simulink model "YMBOX_Control_Core"  (R2024b)
settings: Solver=FixedStepDiscrete  StartTime=0.0  StopTime=3  RelTol=1e-3
PreLoadFcn:
  | run(fullfile(fileparts(get_param(bdroot,'FileName')), 'YMBOX_Deluxe_init.m'));
InitFcn:
  | YMBOX_InitializeModel('core',bdroot);
model workspace (MAT data in the model file):
  KuMDAS_ObserverBuildVariant : Simulink.Parameter (value not decoded)
undefined symbols (not defined in the file or in its folder): CeMDSM_DrvModeIfStart_enum, CeMDSM_DrvModeSpdSens_enum, CeMDSM_DrvModeSpdSmo_enum, CeMDSM_DrvModeTrq_enum, Cf_CONTROL_TASK_TIME_S, KbMDAS_SmoDeadTimeCompEnable_flg, KbMDSA_ActiveInverterCompEnable_flg, KbMDSA_UnifiedVoltageLimitEnable_flg, KbMDSP_DCBusVoltReportFilterEnable_flg, KbMDTM_DAxisPriorityInFW_flg, KbMDTM_FieldWeakeningEnable_flg, KbMDTM_FinalIqAntiWindupEnable_flg, KbMDTM_SensorlessFieldWeakeningEnable_flg, KbMDTM_TorquePriorityBelowBase_flg, KbMDTM_UnifiedConstraintEnable_flg, KfMDAS_ControlCountToElecRad_NULL, KfMDAS_IfAccel_rpms, KfMDAS_IfAlignTime_s, KfMDAS_IfBlendTime_s, KfMDAS_IfSwitchSpd_rpm, KfMDAS_NativeCountToMechRad_NULL, KfMDAS_ObserverExitRatio_NULL, KfMDAS_SlsCtrlPeriod_s, KfMDAS_SlsEAngleInit_rad, KfMDAS_SlsElecSpdMax_rads, KfMDAS_SlsElecSpdMin_rads, KfMDAS_SlsTwoPi_rad, KfMDAS_SmoAngleOffset_rad, KfMDAS_SmoCurrentZohCoefA_NULL, KfMDAS_SmoCurrentZohCoefB_AperV, KfMDAS_SmoDeadTimeCurrentBoundary_A, KfMDAS_SmoDeadTimeDuty_NULL, KfMDAS_SmoDeadTimePolarity_NULL, KfMDAS_SmoDeviceDrop_V, KfMDAS_SmoEmfLpfCoefA_NULL, KfMDAS_SmoEmfLpfCoefB_NULL, KfMDAS_SmoEmfLpfInvPole_s, KfMDAS_SmoErrBoundaryMax_A, KfMDAS_SmoErrBoundarySpan_A, KfMDAS_SmoGainSchedAlpha_NULL, KfMDAS_SmoGainSchedAngleComp_rad, KfMDAS_SmoGainSchedEmfLow_V, KfMDAS_SmoGainSchedInvSpan_PerV, KfMDAS_SmoLdMinusLq_H, KfMDAS_SmoPllKiTs_NULL, KfMDAS_SmoPllKp_NULL, KfMDAS_SmoPllMinEmf_V, KfMDAS_SmoPllSpeedLpfAlpha_NULL, KfMDAS_SmoSlideGainMin_V, KfMDAS_SmoSlideGainSpan_V, KfMDAS_SmoSwitchSpd_rpm, KfMDAS_SmoTotalDelay_s, KfMDCC_DqSoftwareOverCurrentThreshold_A, KfMDCC_PiKcTsId_NULL, KfMDCC_PiKcTsIq_NULL, KfMDCC_PiKiTsId_NULL, KfMDCC_PiKiTsIq_NULL, KfMDCC_PiKpValueId_NULL, KfMDCC_PiKpValueIq_NULL, KfMDCC_PwmFreq_Hz ... (+84)
libraries: YMBOX_SharedMath_Lib x11, spsabctoAlphaBetaZeroLib x1
(part 5 of 8)

== system YMBOX_Control_Core/MDAS/Sensorless_FluxMRAS/Observer_Variant1_SMO/Voltage_AlphaBeta_Reconstruction ==
  VfMDAS_SlsPwmDutyPhaseU_NULL : Inport
  VfMDAS_SlsPwmDutyPhaseV_NULL : Inport  Port=2
  VfMDAS_SlsPwmDutyPhaseW_NULL : Inport  Port=3
  PhaseCurrentU_A : Inport  Port=4
  PhaseCurrentV_A : Inport  Port=5
  PhaseCurrentW_A : Inport  Port=6
  DcBusVoltage_V : Inport  Port=7
  CurrentSignSatU : Saturate  UpperLimit=1  LowerLimit=-1
  CurrentSignSatV : Saturate  UpperLimit=1  LowerLimit=-1
  CurrentSignSatW : Saturate  UpperLimit=1  LowerLimit=-1
  CurrentSignU : Gain  Gain=1/KfMDAS_SmoDeadTimeCurrentBoundary_A
  CurrentSignV : Gain  Gain=1/KfMDAS_SmoDeadTimeCurrentBoundary_A
  CurrentSignW : Gain  Gain=1/KfMDAS_SmoDeadTimeCurrentBoundary_A
  DeadTimeDuty : Gain  Gain=KfMDAS_SmoDeadTimeDuty_NULL
  DeadTimeEnablePolarity : Gain  Gain=KbMDAS_SmoDeadTimeCompEnable_flg*KfMDAS_SmoDeadTimePolarity_NULL
  DeadTimeErrorU : Product  Inputs=**  OutDataTypeStr=single  RndMeth=Nearest  SaturateOnIntegerOverflow=on
  DeadTimeErrorV : Product  Inputs=**  OutDataTypeStr=single  RndMeth=Nearest  SaturateOnIntegerOverflow=on
  DeadTimeErrorW : Product  Inputs=**  OutDataTypeStr=single  RndMeth=Nearest  SaturateOnIntegerOverflow=on
  DeadTimeVoltage : Sum  OutDataTypeStr=single  AccumDataTypeStr=single  RndMeth=Nearest  SaturateOnIntegerOverflow=on
  DeviceDrop : Constant  Value=KfMDAS_SmoDeviceDrop_V  OutDataTypeStr=single
  Duty_alpha_sum : Sum  Inputs=+--
  Duty_beta_sum : Sum  Inputs=+-
  ErrorAlpha : Gain  Gain=2/3
  ErrorAlphaRaw : Sum  Inputs=+--  OutDataTypeStr=single  AccumDataTypeStr=single  RndMeth=Nearest  SaturateOnIntegerOverflow=on
  ErrorBeta : Gain  Gain=sqrt(3)/3
  ErrorBetaRaw : Sum  Inputs=+-  OutDataTypeStr=single  AccumDataTypeStr=single  RndMeth=Nearest  SaturateOnIntegerOverflow=on
  HalfErrorV : Gain  Gain=0.5
  HalfErrorW : Gain  Gain=0.5
  Half_Duty_V : Gain  Gain=0.5
  Half_Duty_W : Gain  Gain=0.5
  Mux_Uab0 : Mux  Inputs=3
  UalphaCompensated : Sum  Inputs=+-  OutDataTypeStr=single  AccumDataTypeStr=single  RndMeth=Nearest  SaturateOnIntegerOverflow=on
  Ualpha_gain : Gain  Gain=2/3
  Ualpha_single : DataTypeConversion  OutDataTypeStr=single  SaturateOnIntegerOverflow=off  RndMeth=Floor
  UbetaCompensated : Sum  Inputs=-+  OutDataTypeStr=single  AccumDataTypeStr=single  RndMeth=Nearest  SaturateOnIntegerOverflow=on
  Ubeta_gain : Gain  Gain=sqrt(3)/3
  Ubeta_single : DataTypeConversion  OutDataTypeStr=single  SaturateOnIntegerOverflow=off  RndMeth=Floor
  VdcDutyAlpha : Product  Inputs=**  OutDataTypeStr=single  RndMeth=Nearest  SaturateOnIntegerOverflow=on
  VdcDutyBeta : Product  Inputs=**  OutDataTypeStr=single  RndMeth=Nearest  SaturateOnIntegerOverflow=on
  Zero_Sequence : Constant  Value=single(0)  OutDataTypeStr=single
  VfMDAS_SlsVoltAlphaBetaZero_V : Outport
  wires:
  Half_Duty_W/1 -> Duty_alpha_sum/3
  Duty_alpha_sum/1 -> VdcDutyAlpha/1
  ErrorAlpha/1 -> UalphaCompensated/2
  VfMDAS_SlsPwmDutyPhaseV_NULL/1 -> Half_Duty_V/1, Duty_beta_sum/1
  DeadTimeErrorV/1 -> HalfErrorV/1, ErrorBetaRaw/1
  DcBusVoltage_V/1 -> VdcDutyBeta/1, DeadTimeDuty/1, VdcDutyAlpha/2
  Mux_Uab0/1 -> VfMDAS_SlsVoltAlphaBetaZero_V/1
  VfMDAS_SlsPwmDutyPhaseU_NULL/1 -> Duty_alpha_sum/1
  DeadTimeEnablePolarity/1 -> DeadTimeErrorU/2, DeadTimeErrorW/1, DeadTimeErrorV/1
  VfMDAS_SlsPwmDutyPhaseW_NULL/1 -> Half_Duty_W/1, Duty_beta_sum/2
  Duty_beta_sum/1 -> VdcDutyBeta/2
  VdcDutyAlpha/1 -> Ualpha_gain/1
  Half_Duty_V/1 -> Duty_alpha_sum/2
  ErrorAlphaRaw/1 -> ErrorAlpha/1
  Ualpha_gain/1 -> UalphaCompensated/1
  PhaseCurrentU_A/1 -> CurrentSignU/1
  DeadTimeErrorU/1 -> ErrorAlphaRaw/1
  PhaseCurrentV_A/1 -> CurrentSignV/1
  DeadTimeDuty/1 -> DeadTimeVoltage/1
  DeviceDrop/1 -> DeadTimeVoltage/2
  VdcDutyBeta/1 -> Ubeta_gain/1
  ErrorBeta/1 -> UbetaCompensated/1
  PhaseCurrentW_A/1 -> CurrentSignW/1
  CurrentSignU/1 -> CurrentSignSatU/1
  CurrentSignV/1 -> CurrentSignSatV/1
  HalfErrorW/1 -> ErrorAlphaRaw/3
  DeadTimeVoltage/1 -> DeadTimeEnablePolarity/1
  CurrentSignW/1 -> CurrentSignSatW/1
  CurrentSignSatU/1 -> DeadTimeErrorU/1
  CurrentSignSatV/1 -> DeadTimeErrorV/2
  CurrentSignSatW/1 -> DeadTimeErrorW/2
  DeadTimeErrorW/1 -> HalfErrorW/1, ErrorBetaRaw/2
  Ubeta_gain/1 -> UbetaCompensated/2
  HalfErrorV/1 -> ErrorAlphaRaw/2
  ErrorBetaRaw/1 -> ErrorBeta/1
  UbetaCompensated/1 -> Ubeta_single/1
  UalphaCompensated/1 -> Ualpha_single/1
  Ubeta_single/1 -> Mux_Uab0/2
  Ualpha_single/1 -> Mux_Uab0/1
  Zero_Sequence/1 -> Mux_Uab0/3

== system YMBOX_Control_Core/MDCC/MDCC_Subsystem/DqSoftwareOverCurrent_Diagnostic/CountWhenDqCurrentExceeded ==
  VuMDCC_DqSoftwareOverCurrentCount_cnt : Inport  OutDataTypeStr=uint8
  Action Port : ActionPort  ActionPortLabel=if(u1 > u2 | u1 ~= u1)
  AssertDqSoftwareOverCurrent : Subsystem  TreatAsAtomicUnit=on
  DqSoftwareOverCurrentConfirmCount : Constant  Value=KuMDCC_DqSoftwareOverCurrentConfirm_cnt
  If : If  NumInputs=2  IfExpression=u1<u2
  IncrementDqSoftwareOverCurrentCount : Subsystem  TreatAsAtomicUnit=on
  VbMDCC_DqSoftwareOverCurrent_flg : Outport  OutputWhenDisabled=reset  InitialOutput=false
  VuMDCC_DqSoftwareOverCurrentCountNew_cnt : Outport  Port=2
  wires:
  DqSoftwareOverCurrentConfirmCount/1 -> If/2
  If/1 -> IncrementDqSoftwareOverCurrentCount/Action
  If/2 -> AssertDqSoftwareOverCurrent/Action
  IncrementDqSoftwareOverCurrentCount/1(VuMDCC_DqSoftwareOverCurrentCountNew_cnt) -> VuMDCC_DqSoftwareOverCurrentCountNew_cnt/1
  AssertDqSoftwareOverCurrent/1(VbMDCC_DqSoftwareOverCurrent_flg) -> VbMDCC_DqSoftwareOverCurrent_flg/1
  VuMDCC_DqSoftwareOverCurrentCount_cnt/1 -> IncrementDqSoftwareOverCurrentCount/1(VuMDCC_DqSoftwareOverCurrentCount_cnt), If/1

== system YMBOX_Control_Core/MDCC/MDCC_Subsystem/DqSoftwareOverCurrent_Diagnostic/CountWhenDqCurrentNormal ==
  VuMDCC_DqSoftwareOverCurrentCount_cnt : Inport
  Action Port : ActionPort  ActionPortLabel=else
  DecrementDqSoftwareOverCurrentCount : Subsystem  TreatAsAtomicUnit=on
  If : If  IfExpression=u1~=0  ShowElse=off
  VuMDCC_DqSoftwareOverCurrentCountNew_cnt : Outport
  wires:
  DecrementDqSoftwareOverCurrentCount/1(VuMDCC_DqSoftwareOverCurrentCountNew_cnt) -> VuMDCC_DqSoftwareOverCurrentCountNew_cnt/1
  If/1 -> DecrementDqSoftwareOverCurrentCount/Action
  VuMDCC_DqSoftwareOverCurrentCount_cnt/1 -> If/1, DecrementDqSoftwareOverCurrentCount/1(VuMDCC_DqSoftwareOverCurrentCount_cnt)

== system YMBOX_Control_Core/MDCC/MDCC_Subsystem/DqSoftwareOverCurrent_Diagnostic/Current_Magnitude_Squared ==
  VfMDCC_DCur_A : Inport
  VfMDCC_QCur_A : Inport  Port=2
  Product : Product
  Product1 : Product
  Sum : Sum
  VfMDCC_CurMagnitudeSq_A2 : Outport
  wires:
  VfMDCC_QCur_A/1 -> Product1/2, Product1/1
  VfMDCC_DCur_A/1 -> Product/1, Product/2
  Product1/1 -> Sum/2
  Product/1 -> Sum/1
  Sum/1 -> VfMDCC_CurMagnitudeSq_A2/1  "VfMDCC_CurMagnitudeSq_A2"

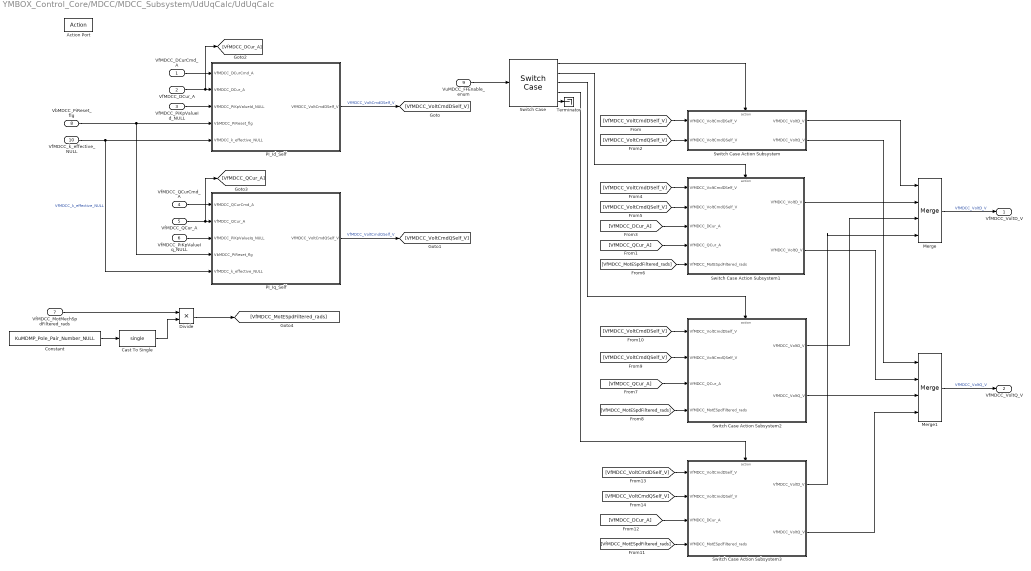
== system YMBOX_Control_Core/MDCC/MDCC_Subsystem/UdUqCalc/UdUqCalc ==
  VfMDCC_DCurCmd_A : Inport
  VfMDCC_DCur_A : Inport  Port=2
  VfMDCC_PiKpValueId_NULL : Inport  Port=3
  VfMDCC_QCurCmd_A : Inport  Port=4
  VfMDCC_QCur_A : Inport  Port=5
  VfMDCC_PiKpValueIq_NULL : Inport  Port=6
  VfMDCC_MotMechSpdFiltered_rads : Inport  Port=7
  VbMDCC_PiReset_flg : Inport  Port=8
  VuMDCC_FFEnable_enum : Inport  Port=9
  VfMDCC_k_effective_NULL : Inport  Port=10
  Action Port : ActionPort  ActionPortLabel=default:
  Cast To Single : DataTypeConversion  OutDataTypeStr=single  SaturateOnIntegerOverflow=off  RndMeth=Floor
  Constant : Constant  Value=KuMDMP_Pole_Pair_Number_NULL
  Divide : Product  Inputs=**
  Merge : Merge  Inputs=4
  Merge1 : Merge  Inputs=4
  PI_Id_Self : Subsystem
  PI_Iq_Self : Subsystem
  Switch Case : SwitchCase  CaseConditions={0,1,2,3}
  Switch Case Action Subsystem : Subsystem  TreatAsAtomicUnit=on
  Switch Case Action Subsystem1 : Subsystem  TreatAsAtomicUnit=on
  Switch Case Action Subsystem2 : Subsystem  TreatAsAtomicUnit=on
  Switch Case Action Subsystem3 : Subsystem  TreatAsAtomicUnit=on
  Terminator : Terminator
  VfMDCC_VoltD_V : Outport
  VfMDCC_VoltQ_V : Outport  Port=2
  wires:
  Cast To Single/1 -> Divide/2
  Constant/1 -> Cast To Single/1
  VfMDCC_MotMechSpdFiltered_rads/1 -> Divide/1
  Divide/1 -> [VfMDCC_MotESpdFiltered_rads]
  [VfMDCC_MotESpdFiltered_rads] -> Switch Case Action Subsystem2/4(VfMDCC_MotESpdFiltered_rads)
  [VfMDCC_MotESpdFiltered_rads] -> Switch Case Action Subsystem1/5(VfMDCC_MotESpdFiltered_rads)
  Switch Case/4 -> Switch Case Action Subsystem3/Action
  Switch Case/3 -> Switch Case Action Subsystem2/Action
  Switch Case/2 -> Switch Case Action Subsystem1/Action
  Switch Case/1 -> Switch Case Action Subsystem/Action
  Switch Case/5 -> Terminator/1
  VfMDCC_k_effective_NULL/1 -> PI_Iq_Self/5(VfMDCC_k_effective_NULL), PI_Id_Self/5(VfMDCC_k_effective_NULL)  "VfMDCC_k_effective_NULL"
  Switch Case Action Subsystem/1(VfMDCC_VoltD_V) -> Merge/1
  Switch Case Action Subsystem1/1(VfMDCC_VoltD_V) -> Merge/2
  Switch Case Action Subsystem2/1(VfMDCC_VoltD_V) -> Merge/3
  Switch Case Action Subsystem3/1(VfMDCC_VoltD_V) -> Merge/4
  Switch Case Action Subsystem/2(VfMDCC_VoltQ_V) -> Merge1/1
  Switch Case Action Subsystem1/2(VfMDCC_VoltQ_V) -> Merge1/2
  Switch Case Action Subsystem2/2(VfMDCC_VoltQ_V) -> Merge1/3
  Switch Case Action Subsystem3/2(VfMDCC_VoltQ_V) -> Merge1/4
  [VfMDCC_VoltCmdQSelf_V] -> Switch Case Action Subsystem3/2(VfMDCC_VoltCmdQSelf_V)
  [VfMDCC_VoltCmdDSelf_V] -> Switch Case Action Subsystem3/1(VfMDCC_VoltCmdDSelf_V)
  [VfMDCC_DCur_A] -> Switch Case Action Subsystem3/3(VfMDCC_DCur_A)
  [VfMDCC_MotESpdFiltered_rads] -> Switch Case Action Subsystem3/4(VfMDCC_MotESpdFiltered_rads)
  [VfMDCC_VoltCmdDSelf_V] -> Switch Case Action Subsystem2/1(VfMDCC_VoltCmdDSelf_V)
  [VfMDCC_VoltCmdQSelf_V] -> Switch Case Action Subsystem2/2(VfMDCC_VoltCmdQSelf_V)
  [VfMDCC_QCur_A] -> Switch Case Action Subsystem2/3(VfMDCC_QCur_A)
  [VfMDCC_VoltCmdQSelf_V] -> Switch Case Action Subsystem1/2(VfMDCC_VoltCmdQSelf_V)
  [VfMDCC_VoltCmdDSelf_V] -> Switch Case Action Subsystem1/1(VfMDCC_VoltCmdDSelf_V)
  [VfMDCC_VoltCmdQSelf_V] -> Switch Case Action Subsystem/2(VfMDCC_VoltCmdQSelf_V)
  [VfMDCC_VoltCmdDSelf_V] -> Switch Case Action Subsystem/1(VfMDCC_VoltCmdDSelf_V)
  PI_Iq_Self/1(VfMDCC_VoltCmdQSelf_V) -> [VfMDCC_VoltCmdQSelf_V]  "VfMDCC_VoltCmdQSelf_V"
  PI_Id_Self/1(VfMDCC_VoltCmdDSelf_V) -> [VfMDCC_VoltCmdDSelf_V]  "VfMDCC_VoltCmdDSelf_V"
  Merge1/1 -> VfMDCC_VoltQ_V/1  "VfMDCC_VoltQ_V"
  Merge/1 -> VfMDCC_VoltD_V/1  "VfMDCC_VoltD_V"
  [VfMDCC_DCur_A] -> Switch Case Action Subsystem1/3(VfMDCC_DCur_A)
  [VfMDCC_QCur_A] -> Switch Case Action Subsystem1/4(VfMDCC_QCur_A)
  VbMDCC_PiReset_flg/1 -> PI_Iq_Self/4(VbMDCC_PiReset_flg), PI_Id_Self/4(VbMDCC_PiReset_flg)
  VuMDCC_FFEnable_enum/1 -> Switch Case/1
  VfMDCC_DCur_A/1 -> [VfMDCC_DCur_A], PI_Id_Self/2(VfMDCC_DCur_A)
  VfMDCC_QCur_A/1 -> [VfMDCC_QCur_A], PI_Iq_Self/2(VfMDCC_QCur_A)
  VfMDCC_PiKpValueIq_NULL/1 -> PI_Iq_Self/3(VfMDCC_PiKpValueIq_NULL)
  VfMDCC_QCurCmd_A/1 -> PI_Iq_Self/1(VfMDCC_QCurCmd_A)
  VfMDCC_PiKpValueId_NULL/1 -> PI_Id_Self/3(VfMDCC_PiKpValueId_NULL)
  VfMDCC_DCurCmd_A/1 -> PI_Id_Self/1(VfMDCC_DCurCmd_A)

== system YMBOX_Control_Core/MDCC/MDCC_Subsystem/UdUqCalc/UdUqCalc2 ==
  VfMDCC_TestUalphaUdId_NULL : Inport
  VfMDCC_TestUbetaUqIq_NULL : Inport  Port=2
  Action Port : ActionPort  ActionPortLabel=case [ 2 ]:
  VfMDCC_VoltD_V : Outport
  VfMDCC_VoltQ_V : Outport  Port=2
  wires:
  VfMDCC_TestUbetaUqIq_NULL/1 -> VfMDCC_VoltQ_V/1
  VfMDCC_TestUalphaUdId_NULL/1 -> VfMDCC_VoltD_V/1

== system YMBOX_Control_Core/MDCC/MDCC_Subsystem/UdUqCalc/UdUqCalc3 ==
  Action Port : ActionPort  ActionPortLabel=case [ 0 1 ]:
  Constant : Constant  Value=0  OutDataTypeStr=single
  Constant1 : Constant  Value=0  OutDataTypeStr=single
  VfMDCC_VoltD_V : Outport
  VfMDCC_VoltQ_V : Outport  Port=2
  wires:
  Constant1/1 -> VfMDCC_VoltQ_V/1
  Constant/1 -> VfMDCC_VoltD_V/1

== system YMBOX_Control_Core/MDSA/Inverter_Nonlinearity_Voltage_Manager/Dq_Compensation_Calculator/Compensation_Limit_Ratio ==
  compSq : Inport  OutDataTypeStr=single
  compMax : Inport  Port=2  OutDataTypeStr=single
  Action Port : ActionPort  ActionPortLabel=if(u1)
  CompMagnitude : YMBOX_SharedMath_Lib/Sqrt_Service  SystemSampleTime=-1  VariantActivationTime=update diagram  AllowFlexibleInterface=on  Latency=0  AutoFrameSizeCalculation=off
  CompScale : Product  Inputs=*/
  scale : Outport
  wires:
  CompScale/1 -> scale/1
  compMax/1 -> CompScale/1
  compSq/1 -> CompMagnitude/1
  CompMagnitude/1 -> CompScale/2

== system YMBOX_Control_Core/MDSA/Inverter_Nonlinearity_Voltage_Manager/Phase_Current_Sign_Manager/Phase_A_Sign_Hold ==
  phaseCurrent : Inport
  posBoundary : Inport  Port=2
  negBoundary : Inport  Port=3
  signHoldCount : Inport  Port=4
  runEnable : Inport  Port=5
  AHit : Logic  Operator=OR  IconShape=distinctive
  AHoldActive : RelationalOperator  Operator=>
  AHoldChoice : Switch  Criteria=u2 ~= 0
  AHoldDec : Sum  Inputs=+-
  AHoldDecFloor : MinMax  Function=max  Inputs=2
  AHoldDelay : UnitDelay  InitialCondition=uint16(0)  SampleTime=-1
  AHoldInit : Switch  Criteria=u2 ~= 0
  AHoldRefresh : Switch  Criteria=u2 ~= 0
  ANeg : RelationalOperator  Operator=<
  APos : RelationalOperator  Operator=>
  ASignD : DataTypeConversion  OutDataTypeStr=single
  ASignDelay : UnitDelay  InitialCondition=int8(0)  SampleTime=-1
  ASignHold : Switch  Criteria=u2 ~= 0
  ASignInit : Switch  Criteria=u2 ~= 0
  ASignNeg : Switch  Criteria=u2 ~= 0
  ASignPos : Switch  Criteria=u2 ~= 0
  NegI8 : Constant  Value=int8(-1)
  OneU16 : Constant  Value=uint16(1)
  PosI8 : Constant  Value=int8(1)
  ZeroI8 : Constant  Value=int8(0)
  ZeroU16 : Constant  Value=uint16(0)
  phaseSign : Outport
  wires:
  ASignD/1 -> phaseSign/1
  ASignInit/1 -> ASignDelay/1, ASignD/1
  ASignPos/1 -> ASignInit/1
  ASignNeg/1 -> ASignPos/3
  ASignHold/1 -> ASignNeg/3
  ASignDelay/1 -> ASignHold/1
  AHoldInit/1 -> AHoldDelay/1
  AHoldRefresh/1 -> AHoldInit/1
  AHoldDec/1 -> AHoldChoice/1
  AHoldActive/1 -> ASignHold/2, AHoldChoice/2
  AHit/1 -> AHoldRefresh/2
  ANeg/1 -> AHit/2, ASignNeg/2
  APos/1 -> AHit/1, ASignPos/2
  negBoundary/1 -> ANeg/2
  phaseCurrent/1 -> APos/1, ANeg/1
  runEnable/1 -> AHoldInit/2, ASignInit/2
  ZeroU16/1 -> AHoldActive/2, AHoldChoice/3, AHoldInit/3
  NegI8/1 -> ASignNeg/1
  PosI8/1 -> ASignPos/1
  ZeroI8/1 -> ASignHold/3, ASignInit/3
  OneU16/1 -> AHoldDec/2, AHoldDecFloor/2
  signHoldCount/1 -> AHoldRefresh/1
  posBoundary/1 -> APos/2
  AHoldDelay/1 -> AHoldActive/1, AHoldDecFloor/1
  AHoldChoice/1 -> AHoldRefresh/3
  AHoldDecFloor/1 -> AHoldDec/1

== system YMBOX_Control_Core/MDSA/Inverter_Nonlinearity_Voltage_Manager/Phase_Current_Sign_Manager/Phase_B_Sign_Hold ==
  phaseCurrent : Inport
  posBoundary : Inport  Port=2
  negBoundary : Inport  Port=3
  signHoldCount : Inport  Port=4
  runEnable : Inport  Port=5
  BHit : Logic  Operator=OR  IconShape=distinctive
  BHoldActive : RelationalOperator  Operator=>
  BHoldChoice : Switch  Criteria=u2 ~= 0
  BHoldDec : Sum  Inputs=+-
  BHoldDecFloor : MinMax  Function=max  Inputs=2
  BHoldDelay : UnitDelay  InitialCondition=uint16(0)  SampleTime=-1
  BHoldInit : Switch  Criteria=u2 ~= 0
  BHoldRefresh : Switch  Criteria=u2 ~= 0
  BNeg : RelationalOperator  Operator=<
  BPos : RelationalOperator  Operator=>
  BSignD : DataTypeConversion  OutDataTypeStr=single
  BSignDelay : UnitDelay  InitialCondition=int8(0)  SampleTime=-1
  BSignHold : Switch  Criteria=u2 ~= 0
  BSignInit : Switch  Criteria=u2 ~= 0
  BSignNeg : Switch  Criteria=u2 ~= 0
  BSignPos : Switch  Criteria=u2 ~= 0
  NegI8 : Constant  Value=int8(-1)
  OneU16 : Constant  Value=uint16(1)
  PosI8 : Constant  Value=int8(1)
  ZeroI8 : Constant  Value=int8(0)
  ZeroU16 : Constant  Value=uint16(0)
  phaseSign : Outport
  wires:
  BSignD/1 -> phaseSign/1
  BSignInit/1 -> BSignDelay/1, BSignD/1
  BSignPos/1 -> BSignInit/1
  BSignNeg/1 -> BSignPos/3
  BSignHold/1 -> BSignNeg/3
  BSignDelay/1 -> BSignHold/1
  BHoldInit/1 -> BHoldDelay/1
  BHoldRefresh/1 -> BHoldInit/1
  BHoldDec/1 -> BHoldChoice/1
  BHoldActive/1 -> BHoldChoice/2, BSignHold/2
  BHit/1 -> BHoldRefresh/2
  BNeg/1 -> BHit/2, BSignNeg/2
  BPos/1 -> BHit/1, BSignPos/2
  negBoundary/1 -> BNeg/2
  phaseCurrent/1 -> BPos/1, BNeg/1
  runEnable/1 -> BHoldInit/2, BSignInit/2
  ZeroU16/1 -> BHoldActive/2, BHoldChoice/3, BHoldInit/3
  NegI8/1 -> BSignNeg/1
  PosI8/1 -> BSignPos/1
  ZeroI8/1 -> BSignHold/3, BSignInit/3
  OneU16/1 -> BHoldDec/2, BHoldDecFloor/2
  signHoldCount/1 -> BHoldRefresh/1
  posBoundary/1 -> BPos/2
  BHoldDelay/1 -> BHoldDecFloor/1, BHoldActive/1
  BHoldChoice/1 -> BHoldRefresh/3
  BHoldDecFloor/1 -> BHoldDec/1

== system YMBOX_Control_Core/MDSA/Inverter_Nonlinearity_Voltage_Manager/Phase_Current_Sign_Manager/Phase_C_Sign_Hold ==
  phaseCurrent : Inport
  posBoundary : Inport  Port=2
  negBoundary : Inport  Port=3
  signHoldCount : Inport  Port=4
  runEnable : Inport  Port=5
  CHit : Logic  Operator=OR  IconShape=distinctive
  CHoldActive : RelationalOperator  Operator=>
  CHoldChoice : Switch  Criteria=u2 ~= 0
  CHoldDec : Sum  Inputs=+-
  CHoldDecFloor : MinMax  Function=max  Inputs=2
  CHoldDelay : UnitDelay  InitialCondition=uint16(0)  SampleTime=-1
  CHoldInit : Switch  Criteria=u2 ~= 0
  CHoldRefresh : Switch  Criteria=u2 ~= 0
  CNeg : RelationalOperator  Operator=<
  CPos : RelationalOperator  Operator=>
  CSignD : DataTypeConversion  OutDataTypeStr=single
  CSignDelay : UnitDelay  InitialCondition=int8(0)  SampleTime=-1
  CSignHold : Switch  Criteria=u2 ~= 0
  CSignInit : Switch  Criteria=u2 ~= 0
  CSignNeg : Switch  Criteria=u2 ~= 0
  CSignPos : Switch  Criteria=u2 ~= 0
  NegI8 : Constant  Value=int8(-1)
  OneU16 : Constant  Value=uint16(1)
  PosI8 : Constant  Value=int8(1)
  ZeroI8 : Constant  Value=int8(0)
  ZeroU16 : Constant  Value=uint16(0)
  phaseSign : Outport
  wires:
  CSignD/1 -> phaseSign/1
  CSignInit/1 -> CSignDelay/1, CSignD/1
  CSignPos/1 -> CSignInit/1
  CSignNeg/1 -> CSignPos/3
  CSignHold/1 -> CSignNeg/3
  CSignDelay/1 -> CSignHold/1
  CHoldInit/1 -> CHoldDelay/1
  CHoldRefresh/1 -> CHoldInit/1
  CHoldDec/1 -> CHoldChoice/1
  CHoldActive/1 -> CHoldChoice/2, CSignHold/2
  CHit/1 -> CHoldRefresh/2
  CNeg/1 -> CHit/2, CSignNeg/2
  CPos/1 -> CHit/1, CSignPos/2
  negBoundary/1 -> CNeg/2
  phaseCurrent/1 -> CPos/1, CNeg/1
  runEnable/1 -> CHoldInit/2, CSignInit/2
  ZeroU16/1 -> CHoldActive/2, CHoldChoice/3, CHoldInit/3
  NegI8/1 -> CSignNeg/1
  PosI8/1 -> CSignPos/1
  ZeroI8/1 -> CSignHold/3, CSignInit/3
  OneU16/1 -> CHoldDec/2, CHoldDecFloor/2
  signHoldCount/1 -> CHoldRefresh/1
  posBoundary/1 -> CPos/2
  CHoldDelay/1 -> CHoldDecFloor/1, CHoldActive/1
  CHoldChoice/1 -> CHoldRefresh/3
  CHoldDecFloor/1 -> CHoldDec/1

== system YMBOX_Control_Core/MDSA/MDSA_Subsystem/PwmOutput/PwmDisable ==
  Action Port : ActionPort  ActionPortLabel=else
  Constant : Constant  Value=0.5  OutDataTypeStr=single
  Constant1 : Constant  Value=0.5  OutDataTypeStr=single
  Constant2 : Constant  Value=0.5  OutDataTypeStr=single
  Constant3 : Constant  Value=0  OutDataTypeStr=single
  VfMDSA_PwmDutyCyclePhaseU_NULL : Outport
  VfMDSA_PwmDutyCyclePhaseV_NULL : Outport  Port=2
  VfMDSA_PwmDutyCyclePhaseW_NULL : Outport  Port=3
  VfMDSA_k_svm_NULL : Outport  Port=4
  wires:
  Constant3/1 -> VfMDSA_k_svm_NULL/1
  Constant/1 -> VfMDSA_PwmDutyCyclePhaseU_NULL/1
  Constant1/1 -> VfMDSA_PwmDutyCyclePhaseV_NULL/1
  Constant2/1 -> VfMDSA_PwmDutyCyclePhaseW_NULL/1

== system YMBOX_Control_Core/MDSA/MDSA_Subsystem/PwmOutput/PwmEnable ==
  VfMDSA_VoltAlpha_V : Inport
  VfMDSA_VoltBeta_V : Inport  Port=2
  VfMDSA_DCBusVolt_V : Inport  Port=3
  Action Port : ActionPort  ActionPortLabel=if(u1)
  SVM : Subsystem  RTWFcnName=vPwm_MDSA_SVM  RTWFileName=MDSA
      settings: RTWSystemCode=Nonreusable function  RTWFcnNameOpts=User specified  RTWFileNameOpts=User specified
  VfMDSA_PwmDutyCyclePhaseU_NULL : Outport
  VfMDSA_PwmDutyCyclePhaseV_NULL : Outport  Port=2
  VfMDSA_PwmDutyCyclePhaseW_NULL : Outport  Port=3
  VfMDSA_k_svm_NULL : Outport  Port=4
  wires:
  SVM/4(VfMDSA_k_svm_NULL) -> VfMDSA_k_svm_NULL/1
  SVM/3(VfMDSA_PwmDutyCyclePhaseW_NULL) -> VfMDSA_PwmDutyCyclePhaseW_NULL/1
  SVM/1(VfMDSA_PwmDutyCyclePhaseU_NULL) -> VfMDSA_PwmDutyCyclePhaseU_NULL/1
  SVM/2(VfMDSA_PwmDutyCyclePhaseV_NULL) -> VfMDSA_PwmDutyCyclePhaseV_NULL/1
  VfMDSA_DCBusVolt_V/1 -> SVM/3(VfMDSA_DCBusVolt_V)
  VfMDSA_VoltAlpha_V/1 -> SVM/1(VfMDSA_VoltAlpha_V)
  VfMDSA_VoltBeta_V/1 -> SVM/2(VfMDSA_VoltBeta_V)

== system YMBOX_Control_Core/MDSA/MDSA_Subsystem/UalphaUbetaCalc/Subsystem ==
  VeMDSA_DrvModeCmd_enum : Inport
  VfMDSA_VoltD_V : Inport  Port=2
  VfMDSA_VoltQ_V : Inport  Port=3
  VfMDSA_MotElecAngle_rad : Inport  Port=4
  VfMDSA_MotElecSpd_rads : Inport  Port=5
  VfMDSA_PwmFreq_Hz : Inport  Port=6
  VfMDSA_TestUalphaUdId_NULL : Inport  Port=7
  VfMDSA_TestUbetaUqIq_NULL : Inport  Port=8
  Action Port : ActionPort  ActionPortLabel=else
  Merge : Merge
  Merge1 : Merge
  Switch Case : SwitchCase  CaseConditions={CeMDSM_DrvModeVoltAB_enum}
  UalphaUbetaCalc1 : Subsystem  TreatAsAtomicUnit=on  RTWFcnName=vPwm_MDSA_UalphaUbetaCalc1  RTWFileName=MDSA
      settings: RTWFcnNameOpts=User specified  RTWFileNameOpts=User specified
  UalphaUbetaCalc2 : Subsystem  TreatAsAtomicUnit=on  RTWFcnName=vPwm_MDSA_UalphaUbetaCalc2  RTWFileName=MDSA
      settings: RTWFcnNameOpts=User specified  RTWFileNameOpts=User specified  RTWMemSecFuncExecute=icache
  VfMDSA_VoltAlpha_V : Outport
  VfMDSA_VoltBeta_V : Outport  Port=2
  wires:
  UalphaUbetaCalc2/2(VfMDSA_VoltBeta_V) -> Merge1/1
  UalphaUbetaCalc1/2(VfMDSA_VoltBeta_V) -> Merge1/2
  UalphaUbetaCalc2/1(VfMDSA_VoltAlpha_V) -> Merge/1
  UalphaUbetaCalc1/1(VfMDSA_VoltAlpha_V) -> Merge/2
  Switch Case/2 -> UalphaUbetaCalc1/Action
  Switch Case/1 -> UalphaUbetaCalc2/Action
  Merge1/1 -> VfMDSA_VoltBeta_V/1
  Merge/1 -> VfMDSA_VoltAlpha_V/1
  VeMDSA_DrvModeCmd_enum/1 -> Switch Case/1
  VfMDSA_PwmFreq_Hz/1 -> UalphaUbetaCalc1/5(VfMDSA_PwmFreq_Hz)
  VfMDSA_MotElecSpd_rads/1 -> UalphaUbetaCalc1/4(VfMDSA_MotElecSpd_rads)
  VfMDSA_MotElecAngle_rad/1 -> UalphaUbetaCalc1/3(VfMDSA_MotElecAngle_rad)
  VfMDSA_VoltQ_V/1 -> UalphaUbetaCalc1/2(VfMDSA_VoltQ_V)  "VfMDSA_VoltQ_V"
  VfMDSA_VoltD_V/1 -> UalphaUbetaCalc1/1(VfMDSA_VoltD_V)  "VfMDSA_VoltD_V"
  VfMDSA_TestUbetaUqIq_NULL/1 -> UalphaUbetaCalc2/2(VfMDSA_TestUbetaUqIq_NULL)
  VfMDSA_TestUalphaUdId_NULL/1 -> UalphaUbetaCalc2/1(VfMDSA_TestUalphaUdId_NULL)

== system YMBOX_Control_Core/MDSA/MDSA_Subsystem/UalphaUbetaCalc/UalphaUbetaCalc2 ==
  Action Port : ActionPort  ActionPortLabel=if(u1 == 0)
  Constant : Constant  Value=0  OutDataTypeStr=Inherit: Inherit via back propagation
  Constant1 : Constant  Value=0  OutDataTypeStr=Inherit: Inherit via back propagation
  VfMDSA_VoltAlpha_V : Outport
  VfMDSA_VoltBeta_V : Outport  Port=2
  wires:
  Constant1/1 -> VfMDSA_VoltBeta_V/1
  Constant/1 -> VfMDSA_VoltAlpha_V/1

== system YMBOX_Control_Core/MDSM/MDSM_ModeManager/MDSM_RouteConfig_Variant/Route_Variant0_SensoredOnly ==
  FalseBoolean : Constant  Value=false  OutDataTypeStr=boolean
  ZeroSingle : Constant  Value=single(0)  OutDataTypeStr=single
  ZeroUint16 : Constant  Value=uint16(0)  OutDataTypeStr=uint16
  VbMDSM_RouteSupported_flg : Outport
  VeMDSM_Stage1Mode_enum : Outport  Port=2
  VbMDSM_Stage1Ready_flg : Outport  Port=3
  VfMDSM_Stage1SwitchSpd_rpm : Outport  Port=4
  VuMDSM_Stage1Acquire_cnt : Outport  Port=5
  VbMDSM_Stage2Enable_flg : Outport  Port=6
  VeMDSM_Stage2Mode_enum : Outport  Port=7
  VbMDSM_Stage2Ready_flg : Outport  Port=8
  VfMDSM_Stage2SwitchSpd_rpm : Outport  Port=9
  VbMDSM_Stage2Fallback_flg : Outport  Port=10
  wires:
  FalseBoolean/1 -> VbMDSM_Stage2Fallback_flg/1, VbMDSM_Stage2Ready_flg/1, VbMDSM_Stage2Enable_flg/1, VbMDSM_Stage1Ready_flg/1, VbMDSM_RouteSupported_flg/1
  ZeroUint16/1 -> VuMDSM_Stage1Acquire_cnt/1, VeMDSM_Stage2Mode_enum/1, VeMDSM_Stage1Mode_enum/1
  ZeroSingle/1 -> VfMDSM_Stage2SwitchSpd_rpm/1, VfMDSM_Stage1SwitchSpd_rpm/1

== system YMBOX_Control_Core/MDSM/MDSM_ModeManager/MDSM_RouteConfig_Variant/Route_Variant1_SMO ==
  VeMDSM_DrvModeReq_enum : Inport
  VbMDAS_SmoReady_flg : Inport  Port=2
  MDSM_ProductRouteConfig : Stateflow chart  TreatAsAtomicUnit=on
  VbMDSM_RouteSupported_flg : Outport
  VeMDSM_Stage1Mode_enum : Outport  Port=2
  VbMDSM_Stage1Ready_flg : Outport  Port=3
  VfMDSM_Stage1SwitchSpd_rpm : Outport  Port=4
  VuMDSM_Stage1Acquire_cnt : Outport  Port=5
  VbMDSM_Stage2Enable_flg : Outport  Port=6
  VeMDSM_Stage2Mode_enum : Outport  Port=7
  VbMDSM_Stage2Ready_flg : Outport  Port=8
  VfMDSM_Stage2SwitchSpd_rpm : Outport  Port=9
  VbMDSM_Stage2Fallback_flg : Outport  Port=10
  wires:
  VeMDSM_DrvModeReq_enum/1 -> MDSM_ProductRouteConfig/1(VeMDSM_DrvModeReq_enum)
  VbMDAS_SmoReady_flg/1 -> MDSM_ProductRouteConfig/2(VbMDAS_SmoReady_flg)
  MDSM_ProductRouteConfig/1(VbMDSM_RouteSupported_flg) -> VbMDSM_RouteSupported_flg/1
  MDSM_ProductRouteConfig/2(VeMDSM_Stage1Mode_enum) -> VeMDSM_Stage1Mode_enum/1
  MDSM_ProductRouteConfig/3(VbMDSM_Stage1Ready_flg) -> VbMDSM_Stage1Ready_flg/1
  MDSM_ProductRouteConfig/4(VfMDSM_Stage1SwitchSpd_rpm) -> VfMDSM_Stage1SwitchSpd_rpm/1
  MDSM_ProductRouteConfig/5(VuMDSM_Stage1Acquire_cnt) -> VuMDSM_Stage1Acquire_cnt/1
  MDSM_ProductRouteConfig/6(VbMDSM_Stage2Enable_flg) -> VbMDSM_Stage2Enable_flg/1
  MDSM_ProductRouteConfig/7(VeMDSM_Stage2Mode_enum) -> VeMDSM_Stage2Mode_enum/1
  MDSM_ProductRouteConfig/8(VbMDSM_Stage2Ready_flg) -> VbMDSM_Stage2Ready_flg/1
  MDSM_ProductRouteConfig/9(VfMDSM_Stage2SwitchSpd_rpm) -> VfMDSM_Stage2SwitchSpd_rpm/1
  MDSM_ProductRouteConfig/10(VbMDSM_Stage2Fallback_flg) -> VbMDSM_Stage2Fallback_flg/1

== system YMBOX_Control_Core/MDSM/MDSM_ModeManager/MDSM_Supervisor_Variant/MDSM_Supervisor_SMO ==
  VeMDSM_DrvModeReq_enum : Inport
  VbMDSM_MCUEnb_flg : Inport  Port=2
  VbMDSM_RouteSupported_flg : Inport  Port=3
  VeMDSM_Stage1Mode_enum : Inport  Port=4
  VbMDSM_Stage1Ready_flg : Inport  Port=5
  VfMDSM_Stage1SwitchSpd_rpm : Inport  Port=6
  VuMDSM_Stage1Acquire_cnt : Inport  Port=7
  VbMDSM_Stage2Enable_flg : Inport  Port=8
  VeMDSM_Stage2Mode_enum : Inport  Port=9
  VbMDSM_Stage2Ready_flg : Inport  Port=10
  VfMDSM_Stage2SwitchSpd_rpm : Inport  Port=11
  VbMDSM_Stage2Fallback_flg : Inport  Port=12
  VfMDSM_TrgtSpd_rpm : Inport  Port=13
  MDSM_GenericSupervisor : Stateflow chart  TreatAsAtomicUnit=on
      settings: AttributesFormatString=|
      | GENERIC TWO-STAGE STATEFLOW
      | I/F -> STAGE1 -> optional STAGE2
      | observer identity is outside the chart
  VeMDSM_DrvModeCmd_enum : Outport
  VbMDTM_PiReset_flg : Outport  Port=2
  VbMDCC_PiReset_flg : Outport  Port=3
  VuMDFM_FFEnable_enum : Outport  Port=4
  wires:
  MDSM_GenericSupervisor/1(VeMDSM_DrvModeCmd_enum) -> VeMDSM_DrvModeCmd_enum/1  "VeMDSM_DrvModeCmd_enum"
  MDSM_GenericSupervisor/2(VbMDTM_PiReset_flg) -> VbMDTM_PiReset_flg/1  "VbMDTM_PiReset_flg"
  VbMDSM_Stage2Fallback_flg/1 -> MDSM_GenericSupervisor/12(VbMDSM_Stage2Fallback_flg)
  VfMDSM_TrgtSpd_rpm/1 -> MDSM_GenericSupervisor/13(VfMDSM_TrgtSpd_rpm)
  MDSM_GenericSupervisor/4(VuMDFM_FFEnable_enum) -> VuMDFM_FFEnable_enum/1  "VuMDFM_FFEnable_enum"
  VfMDSM_Stage2SwitchSpd_rpm/1 -> MDSM_GenericSupervisor/11(VfMDSM_Stage2SwitchSpd_rpm)
  VbMDSM_Stage2Ready_flg/1 -> MDSM_GenericSupervisor/10(VbMDSM_Stage2Ready_flg)
  MDSM_GenericSupervisor/3(VbMDCC_PiReset_flg) -> VbMDCC_PiReset_flg/1  "VbMDCC_PiReset_flg"
  VeMDSM_Stage2Mode_enum/1 -> MDSM_GenericSupervisor/9(VeMDSM_Stage2Mode_enum)
  VuMDSM_Stage1Acquire_cnt/1 -> MDSM_GenericSupervisor/7(VuMDSM_Stage1Acquire_cnt)
  VbMDSM_RouteSupported_flg/1 -> MDSM_GenericSupervisor/3(VbMDSM_RouteSupported_flg)
  VbMDSM_MCUEnb_flg/1 -> MDSM_GenericSupervisor/2(VbMDSM_MCUEnb_flg)
  VeMDSM_Stage1Mode_enum/1 -> MDSM_GenericSupervisor/4(VeMDSM_Stage1Mode_enum)
  VfMDSM_Stage1SwitchSpd_rpm/1 -> MDSM_GenericSupervisor/6(VfMDSM_Stage1SwitchSpd_rpm)
  VbMDSM_Stage1Ready_flg/1 -> MDSM_GenericSupervisor/5(VbMDSM_Stage1Ready_flg)
  VeMDSM_DrvModeReq_enum/1 -> MDSM_GenericSupervisor/1(VeMDSM_DrvModeReq_enum)
  VbMDSM_Stage2Enable_flg/1 -> MDSM_GenericSupervisor/8(VbMDSM_Stage2Enable_flg)

== system YMBOX_Control_Core/MDSM/MDSM_ModeManager/MDSM_Supervisor_Variant/MDSM_Supervisor_SensoredOnly ==
  VeMDSM_DrvModeReq_enum : Inport
  VbMDSM_MCUEnb_flg : Inport  Port=2
  VbMDSM_RouteSupported_flg : Inport  Port=3
  VeMDSM_Stage1Mode_enum : Inport  Port=4
  VbMDSM_Stage1Ready_flg : Inport  Port=5
  VfMDSM_Stage1SwitchSpd_rpm : Inport  Port=6
  VuMDSM_Stage1Acquire_cnt : Inport  Port=7
  VbMDSM_Stage2Enable_flg : Inport  Port=8
  VeMDSM_Stage2Mode_enum : Inport  Port=9
  VbMDSM_Stage2Ready_flg : Inport  Port=10
  VfMDSM_Stage2SwitchSpd_rpm : Inport  Port=11
  VbMDSM_Stage2Fallback_flg : Inport  Port=12
  VfMDSM_TrgtSpd_rpm : Inport  Port=13
  SensoredOnly_Supervisor : MATLAB Function  TreatAsAtomicUnit=on
  TerminateInput03 : Terminator
  TerminateInput04 : Terminator
  TerminateInput05 : Terminator
  TerminateInput06 : Terminator
  TerminateInput07 : Terminator
  TerminateInput08 : Terminator
  TerminateInput09 : Terminator
  TerminateInput{10..13} (4 alike) : Terminator
  VeMDSM_DrvModeCmd_enum : Outport
  VbMDTM_PiReset_flg : Outport  Port=2
  VbMDCC_PiReset_flg : Outport  Port=3
  VuMDFM_FFEnable_enum : Outport  Port=4
  wires:
  VbMDSM_Stage2Enable_flg/1 -> TerminateInput08/1
  VfMDSM_Stage2SwitchSpd_rpm/1 -> TerminateInput11/1
  VbMDSM_RouteSupported_flg/1 -> TerminateInput03/1
  VfMDSM_Stage1SwitchSpd_rpm/1 -> TerminateInput06/1
  VbMDSM_Stage2Ready_flg/1 -> TerminateInput10/1
  VuMDSM_Stage1Acquire_cnt/1 -> TerminateInput07/1
  VbMDSM_Stage2Fallback_flg/1 -> TerminateInput12/1
  VeMDSM_Stage1Mode_enum/1 -> TerminateInput04/1
  VeMDSM_Stage2Mode_enum/1 -> TerminateInput09/1
  VfMDSM_TrgtSpd_rpm/1 -> TerminateInput13/1
  VeMDSM_DrvModeReq_enum/1 -> SensoredOnly_Supervisor/1(modeReq)
  VbMDSM_MCUEnb_flg/1 -> SensoredOnly_Supervisor/2(mcuEnable)
  VbMDSM_Stage1Ready_flg/1 -> TerminateInput05/1
  SensoredOnly_Supervisor/2(mdtmReset) -> VbMDTM_PiReset_flg/1
  SensoredOnly_Supervisor/1(modeCmd) -> VeMDSM_DrvModeCmd_enum/1
  SensoredOnly_Supervisor/4(ffEnable) -> VuMDFM_FFEnable_enum/1
  SensoredOnly_Supervisor/3(mdccReset) -> VbMDCC_PiReset_flg/1

== system YMBOX_Control_Core/MDTM/MDTM/MDTM_SMO/Action_IF_Startup ==
  VfMDTM_SpdCmd_rpm : Inport
  VbMDTM_PiReset_flg : Inport  Port=2
  VfMDTM_ExecutionPeriod_s : Inport  Port=3  OutDataTypeStr=single
  Action Port : ActionPort  ActionPortLabel=case [ 16 ]:
  AlignId_A : Constant  Value=KfMDTM_IfAlignId_A
  AlignTime_s : Constant  Value=KfMDAS_IfAlignTime_s
  BlendTime_s : Constant  Value=KfMDAS_IfBlendTime_s
  IF_Current_Profile : MATLAB Function  TreatAsAtomicUnit=on
  IqSlew_Aps : Constant  Value=KfMDTM_IfIqSlew_Aps
  RunIq_A : Constant  Value=KfMDTM_IfStartIq_A
  Iq : Outport
  Id : Outport  Port=2
  wires:
  VfMDTM_SpdCmd_rpm/1 -> IF_Current_Profile/1(speedCmdRpm)
  VbMDTM_PiReset_flg/1 -> IF_Current_Profile/2(resetFlag)
  AlignTime_s/1 -> IF_Current_Profile/4(alignTime)
  BlendTime_s/1 -> IF_Current_Profile/5(blendTime)
  AlignId_A/1 -> IF_Current_Profile/6(alignId)
  RunIq_A/1 -> IF_Current_Profile/7(runIq)
  IqSlew_Aps/1 -> IF_Current_Profile/8(iqSlew)
  IF_Current_Profile/1(iqCmd) -> Iq/1
  IF_Current_Profile/2(idCmd) -> Id/1
  VfMDTM_ExecutionPeriod_s/1 -> IF_Current_Profile/3(Ts)

== system YMBOX_Control_Core/MDTM/MDTM/MDTM_SMO/SMO_Handover_Current_Comp ==
  iqRaw : Inport  OutDataTypeStr=single
  idRaw : Inport  Port=2  OutDataTypeStr=single
  modeCmd : Inport  Port=3  OutDataTypeStr=uint16
  modeReq : Inport  Port=4  OutDataTypeStr=uint16
  blendWeight : Inport  Port=5  OutDataTypeStr=single
  elecAngleDeltaRad : Inport  Port=6  OutDataTypeStr=single
  ifIq : Inport  Port=7  OutDataTypeStr=single
  measuredSourceId : Inport  Port=8  OutDataTypeStr=single
  measuredSourceIq : Inport  Port=9  OutDataTypeStr=single
  Current_Vector_Crossfade : Subsystem
  Handover_Enable_Logic : Subsystem
  Select_Id_Output : Switch  Criteria=u2 ~= 0
  Select_Iq_Output : Switch  Criteria=u2 ~= 0
  Source_Frame_Rotation : Subsystem
  Target_Frame_Rotation : Subsystem
  Unused_IfIq_Interface : Terminator
  iqOut : Outport  OutDataTypeStr=single
  idOut : Outport  Port=2  OutDataTypeStr=single
  wires:
  Handover_Enable_Logic/1(activeBlend) -> Select_Id_Output/2, Select_Iq_Output/2, Current_Vector_Crossfade/Enable, Source_Frame_Rotation/Enable, Target_Frame_Rotation/Enable
  modeCmd/1 -> Handover_Enable_Logic/1(modeCmd)
  modeReq/1 -> Handover_Enable_Logic/2(modeReq)
  elecAngleDeltaRad/1 -> Target_Frame_Rotation/4(elecAngleDeltaRad), Source_Frame_Rotation/4(elecAngleDeltaRad)
  iqRaw/1 -> Select_Iq_Output/3, Target_Frame_Rotation/2(iqRaw)
  idRaw/1 -> Select_Id_Output/3, Target_Frame_Rotation/1(idRaw)
  Source_Frame_Rotation/2(sourceIq) -> Current_Vector_Crossfade/2(sourceIq)
  Source_Frame_Rotation/1(sourceId) -> Current_Vector_Crossfade/1(sourceId)
  Target_Frame_Rotation/1(targetId) -> Current_Vector_Crossfade/4(targetId)
  Target_Frame_Rotation/2(targetIq) -> Current_Vector_Crossfade/5(targetIq)
  Select_Iq_Output/1 -> iqOut/1
  Current_Vector_Crossfade/2(iqBlend) -> Select_Iq_Output/1
  Current_Vector_Crossfade/1(idBlend) -> Select_Id_Output/1
  Select_Id_Output/1 -> idOut/1
  measuredSourceId/1 -> Source_Frame_Rotation/1(sourceId0)
  measuredSourceIq/1 -> Source_Frame_Rotation/2(sourceIq0)
  ifIq/1 -> Unused_IfIq_Interface/1
  blendWeight/1 -> Source_Frame_Rotation/3(blendWeight), Handover_Enable_Logic/3(blendWeight), Current_Vector_Crossfade/3(currentWeight), Target_Frame_Rotation/3(blendWeight)

== system YMBOX_Control_Core/MDTM/MDTM/MDTM_SMO/SMO_Handover_SeedEstimator ==
  modeCmd : Inport
  modeReq : Inport  Port=2
  blendWeight : Inport  Port=3
  elecAngleDeltaRad : Inport  Port=4
  controlElecAngleRad : Inport  Port=5
  phaseU : Inport  Port=6
  phaseV : Inport  Port=7
  phaseW : Inport  Port=8
  targetSpdRpm : Inport  Port=9
  ifIq : Inport  Port=10
  minDriveIq : Inport  Port=11
  iqLimit : Inport  Port=12
  lpfAlpha : Inport  Port=13
  Enable_Seed_Transform : Logic  AllPortsSameDT=off  OutDataTypeStr=boolean
  Handover_Current_Frame_Transform : Subsystem
  Handover_Seed_State_Manager : MATLAB Function  TreatAsAtomicUnit=on
  Is_Mode_16 : RelationalOperator  Operator===  OutDataTypeStr=boolean  RndMeth=Simplest  InputSameDT=off
  Is_Request_6 : RelationalOperator  Operator===  OutDataTypeStr=boolean  RndMeth=Simplest  InputSameDT=off
  Mode_IF_Startup : Constant  Value=uint16(16)  OutDataTypeStr=uint16
  Request_Product_SMO : Constant  Value=uint16(6)  OutDataTypeStr=uint16
  iqObserverSeed : Outport
  sourceId : Outport  Port=2
  sourceIq : Outport  Port=3
  wires:
  Handover_Seed_State_Manager/3(sourceIq) -> sourceIq/1
  Handover_Seed_State_Manager/2(sourceId) -> sourceId/1
  Handover_Seed_State_Manager/1(iqObserverSeed) -> iqObserverSeed/1
  lpfAlpha/1 -> Handover_Seed_State_Manager/16(lpfAlpha)
  iqLimit/1 -> Handover_Seed_State_Manager/15(iqLimit)
  minDriveIq/1 -> Handover_Seed_State_Manager/14(minDriveIq)
  ifIq/1 -> Handover_Seed_State_Manager/13(ifIq)
  targetSpdRpm/1 -> Handover_Seed_State_Manager/12(targetSpdRpm)
  Handover_Current_Frame_Transform/5(iqObs) -> Handover_Seed_State_Manager/11(iqObs)
  Handover_Current_Frame_Transform/4(iqCtrl) -> Handover_Seed_State_Manager/10(iqCtrl)
  Handover_Current_Frame_Transform/3(idCtrl) -> Handover_Seed_State_Manager/9(idCtrl)
  Handover_Current_Frame_Transform/2(iBeta) -> Handover_Seed_State_Manager/8(iBeta)
  Handover_Current_Frame_Transform/1(iAlpha) -> Handover_Seed_State_Manager/7(iAlpha)
  modeReq/1 -> Handover_Seed_State_Manager/2(modeReq), Is_Request_6/1
  modeCmd/1 -> Handover_Seed_State_Manager/1(modeCmd), Is_Mode_16/1
  phaseW/1 -> Handover_Seed_State_Manager/5(phaseW), Handover_Current_Frame_Transform/6(phaseW)
  phaseV/1 -> Handover_Seed_State_Manager/4(phaseV), Handover_Current_Frame_Transform/5(phaseV)
  phaseU/1 -> Handover_Seed_State_Manager/3(phaseU), Handover_Current_Frame_Transform/4(phaseU)
  controlElecAngleRad/1 -> Handover_Current_Frame_Transform/3(controlElecAngleRad)
  elecAngleDeltaRad/1 -> Handover_Seed_State_Manager/6(elecAngleDeltaRad), Handover_Current_Frame_Transform/2(elecAngleDeltaRad)
  blendWeight/1 -> Handover_Current_Frame_Transform/1(blendWeight)
  Mode_IF_Startup/1 -> Is_Mode_16/2
  Request_Product_SMO/1 -> Is_Request_6/2
  Is_Mode_16/1 -> Enable_Seed_Transform/1
  Is_Request_6/1 -> Enable_Seed_Transform/2
  Enable_Seed_Transform/1 -> Handover_Current_Frame_Transform/Enable

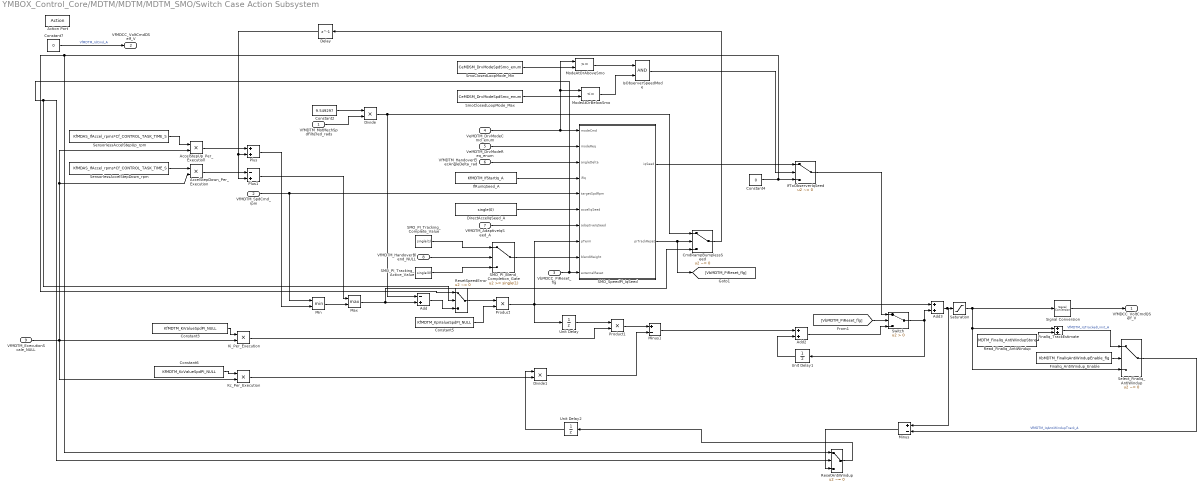
== system YMBOX_Control_Core/MDTM/MDTM/MDTM_SMO/Switch Case Action Subsystem ==
  VfMDTM_MotMechSpdFiltered_rads : Inport
  VfMDTM_SpdCmd_rpm : Inport  Port=2
  VbMDCC_PiReset_flg : Inport  Port=3
  VeMDTM_DrvModeCmd_enum : Inport  Port=4
  VeMDTM_DrvModeReq_enum : Inport  Port=5
  VfMDTM_HandoverElecAngleDelta_rad : Inport  Port=6
  VfMDTM_AdaptiveIqSeed_A : Inport  Port=7
  VfMDTM_HandoverBlend_NULL : Inport  Port=8
  VfMDTM_ExecutionScale_NULL : Inport  Port=9  OutDataTypeStr=single
  Action Port : ActionPort  InitializeStates=reset  ActionPortLabel=case [ 4 17 ]:
  AccelStepDown_Per_Execution : Product  Inputs=**
  AccelStepUp_Per_Execution : Product  Inputs=**
  Add : Sum  Inputs=-+
  Add2 : Sum  OutDataTypeStr=single
  Add3 : Sum
  CmdRampBumplessSeed : Switch  Criteria=u2 ~= 0  Threshold=0.5  SaturateOnIntegerOverflow=off  InputSameDT=off
  Constant2 : Constant  Value=9.549297  OutDataTypeStr=single
  Constant3 : Constant  Value=KfMDTM_KiValueSpdPI_NULL
  Constant4 : Constant  Value=0  OutDataTypeStr=single
  Constant5 : Constant  Value=KfMDTM_KpValueSpdPI_NULL
  Constant6 : Constant  Value=KfMDTM_KcValueSpdPI_NULL
  Constant7 : Constant  Value=0  OutDataTypeStr=single
  Delay : Delay  DelayLength=1
  DirectAccelIqSeed_A : Constant  Description=No forced acceleration-current floor during measured-current PI tracking. Direction guard and current limits remain active.  Value=single(0)
  Divide : Product  Inputs=**
  Divide1 : Product  Inputs=**
  FinalIq_AntiWindup_Enable : Constant  Value=KbMDTM_FinalIqAntiWindupEnable_flg
  FinalIq_TrackEstimate : Sum
  IfRunIqSeed_A : Constant  Value=KfMDTM_IfStartIq_A
  IfToObserverIqSeed : Switch  Criteria=u2 ~= 0  Threshold=0.5  SaturateOnIntegerOverflow=off  InputSameDT=off
  IsObserverSpeedMode : Logic  AllPortsSameDT=off  OutDataTypeStr=boolean
  Kc_Per_Execution : Product  Inputs=**
  Ki_Per_Execution : Product  Inputs=**
  Max : MinMax  Function=max  Inputs=2  OutDataTypeStr=single
  Min : MinMax  Inputs=2  OutDataTypeStr=single
  Minus : Sum  Inputs=+-
  Minus1 : Sum  Inputs=+-
  ModeAtOrAboveSmo : RelationalOperator  OutDataTypeStr=boolean  RndMeth=Simplest  InputSameDT=off
  ModeAtOrBelowSmo : RelationalOperator  Operator=<=  OutDataTypeStr=boolean  RndMeth=Simplest  InputSameDT=off
  Plus : Sum
  Plus1 : Sum  Inputs=-+
  Product : Product
  Product1 : Product  RndMeth=Zero
  Read_FinalIq_AntiWindup : DataStoreRead  DataStoreName=MDTM_FinalIq_AntiWindupStore  IndexOptions=Index vector (dialog)  Indices=1  OutputSizes=1
  ResetAntiWindup : Switch  Criteria=u2 ~= 0
  ResetSpeedError : Switch  Criteria=u2 ~= 0
  SMO_PI_Blend_Completion_Gate : Switch  Threshold=single(1)  OutDataTypeStr=single
  SMO_PI_Tracking_Active_Value : Constant  Value=single(0)  OutDataTypeStr=single
  SMO_PI_Tracking_Complete_Value : Constant  Value=single(1)  OutDataTypeStr=single
  SMO_SpeedPI_IqSeed : MATLAB Function  TreatAsAtomicUnit=on
      settings: AttributesFormatString=BUMPLESS SMO SPEED PI\nIint = Iq target - P\ntrack until actual blend = 100%
  Saturation : Saturate  UpperLimit=KfMDTM_IqCmdMax_A  LowerLimit=KfMDTM_IqCmdMin_A  OutDataTypeStr=single
  Select_FinalIq_AntiWindup : Switch  Criteria=u2 ~= 0
  SensorlessAccelStepDown_rpm : Constant  Value=KfMDAS_IfAccel_rpms*Cf_CONTROL_TASK_TIME_S
  SensorlessAccelStepUp_rpm : Constant  Value=KfMDAS_IfAccel_rpms*Cf_CONTROL_TASK_TIME_S
  Signal Conversion : SignalConversion  OverrideOpt=off
  SmoClosedLoopMode_Max : Constant  Value=CeMDSM_DrvModeSpdSmo_enum  OutDataTypeStr=uint16
  SmoClosedLoopMode_Min : Constant  Value=CeMDSM_DrvModeSpdSmo_enum  OutDataTypeStr=uint16
  Switch : Switch  Criteria=u2 > Threshold  SaturateOnIntegerOverflow=off  InputSameDT=off
  Unit Delay : UnitDelay  SampleTime=-1  HasFrameUpgradeWarning=on
  Unit Delay1 : UnitDelay  SampleTime=-1  HasFrameUpgradeWarning=on
  Unit Delay2 : UnitDelay  SampleTime=-1  HasFrameUpgradeWarning=on
  VfMDCC_VoltCmdQSelf_V : Outport
  VfMDCC_VoltCmdDSelf_V : Outport  Port=2
  wires:
  Constant7/1 -> VfMDCC_VoltCmdDSelf_V/1  "VfMDTM_IdCmd_A"
  AccelStepDown_Per_Execution/1 -> Plus1/1
  Constant6/1 -> Kc_Per_Execution/1
  SensorlessAccelStepUp_rpm/1 -> AccelStepUp_Per_Execution/1
  Max/1 -> Add/2, CmdRampBumplessSeed/3
  SensorlessAccelStepDown_rpm/1 -> AccelStepDown_Per_Execution/1
  SMO_PI_Tracking_Active_Value/1 -> SMO_PI_Blend_Completion_Gate/3
  VfMDTM_ExecutionScale_NULL/1 -> AccelStepUp_Per_Execution/2, AccelStepDown_Per_Execution/2, Ki_Per_Execution/2, Kc_Per_Execution/2
  Constant3/1 -> Ki_Per_Execution/1
  AccelStepUp_Per_Execution/1 -> Plus/1
  Select_FinalIq_AntiWindup/1 -> Minus/2  "VfMDTM_IqAntiWindupTrack_A"
  Ki_Per_Execution/1 -> Product1/2
  Saturation/1 -> Signal Conversion/1, FinalIq_TrackEstimate/1, Select_FinalIq_AntiWindup/3
  Kc_Per_Execution/1 -> Divide1/2
  Plus/1 -> Min/2
  VfMDTM_MotMechSpdFiltered_rads/1 -> Divide/2
  Plus1/1 -> Max/1
  VfMDTM_SpdCmd_rpm/1 -> SMO_SpeedPI_IqSeed/5(targetSpdRpm), Min/1
  Delay/1 -> Plus1/2, Plus/2
  Constant2/1 -> Divide/1
  Min/1 -> Max/2
  Divide/1 -> Add/1, CmdRampBumplessSeed/1
  SMO_PI_Tracking_Complete_Value/1 -> SMO_PI_Blend_Completion_Gate/1
  SMO_PI_Blend_Completion_Gate/1 -> SMO_SpeedPI_IqSeed/9(blendWeight)
  VfMDTM_HandoverBlend_NULL/1 -> SMO_PI_Blend_Completion_Gate/2
  Add/1 -> ResetSpeedError/3
  Constant5/1 -> Product/2
  Product1/1 -> Minus1/1
  VeMDTM_DrvModeReq_enum/1 -> SMO_SpeedPI_IqSeed/2(modeReq)
  Read_FinalIq_AntiWindup/1 -> FinalIq_TrackEstimate/2
  VfMDTM_HandoverElecAngleDelta_rad/1 -> SMO_SpeedPI_IqSeed/3(angleDelta)
  IfRunIqSeed_A/1 -> SMO_SpeedPI_IqSeed/4(ifIq)
  DirectAccelIqSeed_A/1 -> SMO_SpeedPI_IqSeed/6(accelIqSeed)
  VfMDTM_AdaptiveIqSeed_A/1 -> SMO_SpeedPI_IqSeed/7(adaptiveIqSeed)
  Product/1 -> SMO_SpeedPI_IqSeed/8(pTerm), Add3/1, Unit Delay/1
  VbMDCC_PiReset_flg/1 -> ResetAntiWindup/2, ResetSpeedError/2, SMO_SpeedPI_IqSeed/10(externalReset)
  VeMDTM_DrvModeCmd_enum/1 -> SMO_SpeedPI_IqSeed/1(modeCmd), ModeAtOrAboveSmo/1, ModeAtOrBelowSmo/1
  Minus/1 -> ResetAntiWindup/3
  SmoClosedLoopMode_Min/1 -> ModeAtOrAboveSmo/2
  SmoClosedLoopMode_Max/1 -> ModeAtOrBelowSmo/2
  Unit Delay2/1 -> Divide1/1
  SMO_SpeedPI_IqSeed/1(iqSeed) -> IfToObserverIqSeed/1
  Add2/1 -> Switch/3
  SMO_SpeedPI_IqSeed/2(piTrackReset) -> [VbMDTM_PiReset_flg], CmdRampBumplessSeed/2
  ModeAtOrAboveSmo/1 -> IsObserverSpeedMode/1
  Unit Delay/1 -> Product1/1
  ModeAtOrBelowSmo/1 -> IsObserverSpeedMode/2
  CmdRampBumplessSeed/1 -> Delay/1
  Divide1/1 -> Minus1/2
  IsObserverSpeedMode/1 -> IfToObserverIqSeed/2
  Constant4/1 -> ResetSpeedError/1, ResetAntiWindup/1, IfToObserverIqSeed/3
  Switch/1 -> Unit Delay1/1, Add3/2
  Minus1/1 -> Add2/1
  IfToObserverIqSeed/1 -> Switch/1
  Unit Delay1/1 -> Add2/2
  [VbMDTM_PiReset_flg] -> Switch/2
  Add3/1 -> Minus/1, Saturation/1
  Signal Conversion/1 -> VfMDCC_VoltCmdQSelf_V/1
  FinalIq_TrackEstimate/1 -> Select_FinalIq_AntiWindup/1  "VfMDTM_IqTrackedLimit_A"
  FinalIq_AntiWindup_Enable/1 -> Select_FinalIq_AntiWindup/2
  ResetSpeedError/1 -> Product/1
  ResetAntiWindup/1 -> Unit Delay2/1

== system YMBOX_Control_Core/MDTM/MDTM/MDTM_SMO/Switch Case Action Subsystem1 ==
  VfMDCC_TestUalphaUdId_NULL : Inport
  VfMDTM_TestUbetaUqIq_NULL : Inport  Port=2
  Action Port : ActionPort  ActionPortLabel=case [ 3 ]:
  Iq : Outport
  Id : Outport  Port=2
  wires:
  VfMDCC_TestUalphaUdId_NULL/1 -> Id/1
  VfMDTM_TestUbetaUqIq_NULL/1 -> Iq/1

== system YMBOX_Control_Core/MDTM/MDTM/MDTM_SMO/Switch Case Action Subsystem2 ==
  VfMDTM_TrqCmd_Nm : Inport
  Action Port : ActionPort  ActionPortLabel=case [ 5 ]:
  Constant7 : Constant  Value=0  OutDataTypeStr=single
  Gain : Gain  Gain=KfMDTM_Trq2Iq_NULL
  Iq : Outport
  Id : Outport  Port=2
  wires:
  VfMDTM_TrqCmd_Nm/1 -> Gain/1
  Constant7/1 -> Id/1  "VfMDTM_IdCmd_A"
  Gain/1 -> Iq/1
